simulink model "r2_b16a4x512f"  (R2012b)
settings: Solver=VariableStepDiscrete  SolverMode=SingleTasking  StartTime=0.0  StopTime=1  RelTol=1e-3
undefined symbols (not defined in the file): fft_stages, n_bits_ants, n_bits_xengs
libraries: xbsIndex_r4 x27410, casper_library_misc x230, xbsReplacements_r4 x24, casper_library_delays x8, xps_library x5, casper_library_communications x4
(part 100 of 229)

== system r2_b16a4x512f/sys0/vacc/zeros/bus_create ==
  in1 : Inport
  in2 : Inport  Port=2
  in3 : Inport  Port=3
  in4 : Inport  Port=4
  in5 : Inport  Port=5
  in6 : Inport  Port=6
  in7 : Inport  Port=7
  in8 : Inport  Port=8
  in9 : Inport  Port=9
  in10 : Inport  Port=10
  in11 : Inport  Port=11
  in12 : Inport  Port=12
  in13 : Inport  Port=13
  in14 : Inport  Port=14
  in15 : Inport  Port=15
  in16 : Inport  Port=16
  in17 : Inport  Port=17
  in18 : Inport  Port=18
  in19 : Inport  Port=19
  concatenate : xbsIndex_r4/Concat  num_inputs=19  dbl_ovrd=off  block_type=concat
  reinterpret{1..19} (19 alike) : xbsIndex_r4/Reinterpret  force_arith_type=on  arith_type=Unsigned  force_bin_pt=on  bin_pt=0  block_type=reinterpret
      reinterpret1 settings: infoedit="Changes signal type without altering the binary representation.   You can changed the signal between signed and unsigned, and relocate the binary point.<br><br>Hardware notes: In hardware this block costs nothing.<br><br>Example:  Suppose the input is 6 bits wide, signed, with 2 fractional bits, and the output is forced to unsigned with 0 fractional bits.  Then an input of -2.0 (1110.00 in binary 2's complement) becomes an output of 56 (111000 in binary)."
  bus_out : Outport
  wires:
  concatenate/1 -> bus_out/1
  in1/1 -> reinterpret1/1
  reinterpret1/1 -> concatenate/1
  in2/1 -> reinterpret2/1
  reinterpret2/1 -> concatenate/2
  in3/1 -> reinterpret3/1
  reinterpret3/1 -> concatenate/3
  in4/1 -> reinterpret4/1
  reinterpret4/1 -> concatenate/4
  in5/1 -> reinterpret5/1
  reinterpret5/1 -> concatenate/5
  in6/1 -> reinterpret6/1
  reinterpret6/1 -> concatenate/6
  in7/1 -> reinterpret7/1
  reinterpret7/1 -> concatenate/7
  in8/1 -> reinterpret8/1
  reinterpret8/1 -> concatenate/8
  in9/1 -> reinterpret9/1
  reinterpret9/1 -> concatenate/9
  in10/1 -> reinterpret10/1
  reinterpret10/1 -> concatenate/10
  in11/1 -> reinterpret11/1
  reinterpret11/1 -> concatenate/11
  in12/1 -> reinterpret12/1
  reinterpret12/1 -> concatenate/12
  in13/1 -> reinterpret13/1
  reinterpret13/1 -> concatenate/13
  in14/1 -> reinterpret14/1
  reinterpret14/1 -> concatenate/14
  in15/1 -> reinterpret15/1
  reinterpret15/1 -> concatenate/15
  in16/1 -> reinterpret16/1
  reinterpret16/1 -> concatenate/16
  in17/1 -> reinterpret17/1
  reinterpret17/1 -> concatenate/17
  in18/1 -> reinterpret18/1
  reinterpret18/1 -> concatenate/18
  in19/1 -> reinterpret19/1
  reinterpret19/1 -> concatenate/19

== system r2_b16a4x512f/sys0/vacc_tvg0/bus_replicate/bussify ==
  in1 : Inport
  in2 : Inport  Port=2
  concatenate : xbsIndex_r4/Concat  num_inputs=2  dbl_ovrd=off  block_type=concat
  reinterpret1 : xbsIndex_r4/Reinterpret  force_arith_type=on  arith_type=Unsigned  force_bin_pt=on  bin_pt=0  block_type=reinterpret
      settings: infoedit="Changes signal type without altering the binary representation.   You can changed the signal between signed and unsigned, and relocate the binary point.<br><br>Hardware notes: In hardware this block costs nothing.<br><br>Example:  Suppose the input is 6 bits wide, signed, with 2 fractional bits, and the output is forced to unsigned with 0 fractional bits.  Then an input of -2.0 (1110.00 in binary 2's complement) becomes an output of 56 (111000 in binary)."
  reinterpret2 : xbsIndex_r4/Reinterpret  force_arith_type=on  arith_type=Unsigned  force_bin_pt=on  bin_pt=0  block_type=reinterpret
      settings: infoedit="Changes signal type without altering the binary representation.   You can changed the signal between signed and unsigned, and relocate the binary point.<br><br>Hardware notes: In hardware this block costs nothing.<br><br>Example:  Suppose the input is 6 bits wide, signed, with 2 fractional bits, and the output is forced to unsigned with 0 fractional bits.  Then an input of -2.0 (1110.00 in binary 2's complement) becomes an output of 56 (111000 in binary)."
  bus_out : Outport
  wires:
  concatenate/1 -> bus_out/1
  in1/1 -> reinterpret1/1
  reinterpret1/1 -> concatenate/1
  in2/1 -> reinterpret2/1
  reinterpret2/1 -> concatenate/2

== system r2_b16a4x512f/sys0/vacc_tvg0/bus_replicate1/bussify ==
  in1 : Inport
  in2 : Inport  Port=2
  concatenate : xbsIndex_r4/Concat  num_inputs=2  dbl_ovrd=off  block_type=concat
  reinterpret1 : xbsIndex_r4/Reinterpret  force_arith_type=on  arith_type=Unsigned  force_bin_pt=on  bin_pt=0  block_type=reinterpret
      settings: infoedit="Changes signal type without altering the binary representation.   You can changed the signal between signed and unsigned, and relocate the binary point.<br><br>Hardware notes: In hardware this block costs nothing.<br><br>Example:  Suppose the input is 6 bits wide, signed, with 2 fractional bits, and the output is forced to unsigned with 0 fractional bits.  Then an input of -2.0 (1110.00 in binary 2's complement) becomes an output of 56 (111000 in binary)."
  reinterpret2 : xbsIndex_r4/Reinterpret  force_arith_type=on  arith_type=Unsigned  force_bin_pt=on  bin_pt=0  block_type=reinterpret
      settings: infoedit="Changes signal type without altering the binary representation.   You can changed the signal between signed and unsigned, and relocate the binary point.<br><br>Hardware notes: In hardware this block costs nothing.<br><br>Example:  Suppose the input is 6 bits wide, signed, with 2 fractional bits, and the output is forced to unsigned with 0 fractional bits.  Then an input of -2.0 (1110.00 in binary 2's complement) becomes an output of 56 (111000 in binary)."
  bus_out : Outport
  wires:
  reinterpret2/1 -> concatenate/2
  in2/1 -> reinterpret2/1
  reinterpret1/1 -> concatenate/1
  in1/1 -> reinterpret1/1
  concatenate/1 -> bus_out/1

== system r2_b16a4x512f/sys0/vacc_tvg0/generate_pulses/edge_detect ==
  in : Inport
  Delay : xbsIndex_r4/Delay  rst=off  infoeditControl=Selection of Reset will increase slice count due to use of real FFs and instead of SRLs  en=off  latency=1  dbl_ovrd=off  reg_retiming=on  block_type=delay
      settings: xl_area=[0, 0, 0, 0, 0, 0, 0]
  Inverter : xbsIndex_r4/Inverter  en=off  latency=0  dbl_ovrd=off  block_type=inv
      settings: xl_area=[0, 0, 0, 0, 0, 0, 0]
  edge_op : xbsIndex_r4/Logical  logical_function=NOR  inputs=2  en=off  latency=0  precision=Full  arith_type=Unsigned  n_bits=8  bin_pt=2  align_bp=on  dbl_ovrd=off  block_type=logical
      settings: xl_area=[0, 0, 0, 0, 0, 0, 0]
  out : Outport
  wires:
  Delay/1 -> edge_op/2
  in/1 -> Delay/1, Inverter/1
  edge_op/1 -> out/1
  Inverter/1 -> edge_op/1

== system r2_b16a4x512f/sys0/vacc_tvg0/generate_pulses/edge_detect1 ==
  in : Inport
  Delay : xbsIndex_r4/Delay  rst=off  infoeditControl=Selection of Reset will increase slice count due to use of real FFs and instead of SRLs  en=off  latency=1  dbl_ovrd=off  reg_retiming=on  block_type=delay
      settings: xl_area=[0, 0, 0, 0, 0, 0, 0]
  Inverter : xbsIndex_r4/Inverter  en=off  latency=0  dbl_ovrd=off  block_type=inv
      settings: xl_area=[0, 0, 0, 0, 0, 0, 0]
  edge_op : xbsIndex_r4/Logical  logical_function=XNOR  inputs=2  en=off  latency=0  precision=Full  arith_type=Unsigned  n_bits=8  bin_pt=2  align_bp=on  dbl_ovrd=off  block_type=logical
      settings: xl_area=[0, 0, 0, 0, 0, 0, 0]
  out : Outport
  wires:
  Inverter/1 -> edge_op/1
  edge_op/1 -> out/1
  in/1 -> Inverter/1, Delay/1
  Delay/1 -> edge_op/2

== system r2_b16a4x512f/sys0/vacc_tvg0/ins_counter/bus_replicate1 ==
  in : Inport
  bussify : Subsystem  AncestorBlock=casper_library_flow_control/bus_create  mask(bus_create){inputNum=2}
      mask prompts: inputNum "Number of inputs:"
      mask init:
      | bus_create_init(gcb,...
      |     'inputNum', inputNum);
  out : Outport
  wires:
  in/1 -> bussify/1(in1), bussify/2(in2)
  bussify/1(bus_out) -> out/1

== system r2_b16a4x512f/sys0/xeng/auto_tap/delay ==
  din : Inport
  constant : xbsIndex_r4/Constant  const=1  gui_display_data_type=Fixed-point  arith_type=Boolean  n_bits=16  bin_pt=14  preci_type=Single  exp_width=8  frac_width=24  explicit_period=on  period=1  equ=P=C  opselect=C  inp2=PCIN>>17  opr=+  inp1=P  carry=CIN  dbl_ovrd=off  block_type=constant
  counter : xbsIndex_r4/Counter  cnt_type=Count Limited  cnt_to=DelayLen - bram_latency - 1  operation=Up  start_count=0  cnt_by_val=1  arith_type=Unsigned  n_bits=11  bin_pt=0  load_pin=off  rst=off  en=off  explicit_period=on  period=1  dbl_ovrd=off  use_behavioral_HDL=off  implementation=Fabric  use_rpm=off  block_type=counter
  ram : xbsIndex_r4/Single Port RAM  depth=2048  initVector=0  distributed_mem=Block RAM  write_mode=Read Before Write  rst=off  init_reg=0  en=off  latency=bram_latency  dbl_ovrd=off  optimize=Area  block_type=spram
  dout : Outport
  wires:
  counter/1 -> ram/1
  din/1 -> ram/2
  constant/1 -> ram/3
  ram/1 -> dout/1

== system r2_b16a4x512f/sys0/xeng/auto_tap/dual_pol_cmac ==
  a1 : Inport
  a2 : Inport  Port=2
  acc_in : Inport  Port=3
  sync : Inport  Port=4
  valid_in : Inport  Port=5
  Concat : xbsIndex_r4/Concat  num_inputs=4  dbl_ovrd=off  block_type=concat
      settings: block_version=9.2.01
  Constant1 : xbsIndex_r4/Constant  const=0  gui_display_data_type=Fixed-point  arith_type=Unsigned  n_bits=1  bin_pt=0  preci_type=Single  exp_width=8  frac_width=24  explicit_period=on  period=1  equ=P=C  opselect=C  inp2=PCIN>>17  opr=+  inp1=P  carry=CIN  dbl_ovrd=off  block_type=constant
      settings: block_version=9.2.01
  Constant2 : xbsIndex_r4/Constant  const=0  gui_display_data_type=Fixed-point  arith_type=Unsigned  n_bits=1  bin_pt=0  preci_type=Single  exp_width=8  frac_width=24  explicit_period=on  period=1  equ=P=C  opselect=C  inp2=PCIN>>17  opr=+  inp1=P  carry=CIN  dbl_ovrd=off  block_type=constant
      settings: block_version=9.2.01
  Constant4 : xbsIndex_r4/Constant  const=0  gui_display_data_type=Fixed-point  arith_type=Unsigned  n_bits=1  bin_pt=0  preci_type=Single  exp_width=8  frac_width=24  explicit_period=on  period=1  equ=P=C  opselect=C  inp2=PCIN>>17  opr=+  inp1=P  carry=CIN  dbl_ovrd=off  block_type=constant
      settings: block_version=9.2.01
  Slice{,1,6,10} (4 alike) : xbsIndex_r4/Slice  nbits=2*n_bits  boolean_output=off  mode=Upper Bit Location + Width  bit1=0  base1=MSB of Input  bit0=0  base0=LSB of Input  dbl_ovrd=off  block_type=slice
      Slice settings: infoedit="Extracts a given range of bits from each input sample and presents it at the output.  The output type is ordinarily unsigned with binary point at zero, but can be Boolean when the slice is one bit wide.<P><P>Hardware notes: In hardware this block costs nothing."  block_version=9.2.01
      Slice1 settings: infoedit="Extracts a given range of bits from each input sample and presents it at the output.  The output type is ordinarily unsigned with binary point at zero, but can be Boolean when the slice is one bit wide.<P><P>Hardware notes: In hardware this block costs nothing."  block_version=9.2.01
      Slice10 settings: block_version=9.2.01
      Slice6 settings: infoedit="Extracts a given range of bits from each input sample and presents it at the output.  The output type is ordinarily unsigned with binary point at zero, but can be Boolean when the slice is one bit wide.<P><P>Hardware notes: In hardware this block costs nothing."  block_version=9.2.01
  Slice11 : xbsIndex_r4/Slice  nbits=2*n_bits_out  boolean_output=off  mode=Upper Bit Location + Width  bit1=-6*n_bits_out  base1=MSB of Input  bit0=0  base0=LSB of Input  dbl_ovrd=off  block_type=slice
      settings: infoedit="Extracts a given range of bits from each input sample and presents it at the output.  The output type is ordinarily unsigned with binary point at zero, but can be Boolean when the slice is one bit wide.<P><P>Hardware notes: In hardware this block costs nothing."  block_version=9.2.01
  Slice2 : xbsIndex_r4/Slice  nbits=2*n_bits_out  boolean_output=off  mode=Upper Bit Location + Width  bit1=0  base1=MSB of Input  bit0=0  base0=LSB of Input  dbl_ovrd=off  block_type=slice
      settings: infoedit="Extracts a given range of bits from each input sample and presents it at the output.  The output type is ordinarily unsigned with binary point at zero, but can be Boolean when the slice is one bit wide.<P><P>Hardware notes: In hardware this block costs nothing."  block_version=9.2.01
  Slice{3..4,7,9} (4 alike) : xbsIndex_r4/Slice  nbits=2*n_bits  boolean_output=off  mode=Upper Bit Location + Width  bit1=-2*n_bits  base1=MSB of Input  bit0=0  base0=LSB of Input  dbl_ovrd=off  block_type=slice
      Slice3 settings: infoedit="Extracts a given range of bits from each input sample and presents it at the output.  The output type is ordinarily unsigned with binary point at zero, but can be Boolean when the slice is one bit wide.<P><P>Hardware notes: In hardware this block costs nothing."  block_version=9.2.01
      Slice4 settings: infoedit="Extracts a given range of bits from each input sample and presents it at the output.  The output type is ordinarily unsigned with binary point at zero, but can be Boolean when the slice is one bit wide.<P><P>Hardware notes: In hardware this block costs nothing."  block_version=9.2.01
      Slice7 settings: infoedit="Extracts a given range of bits from each input sample and presents it at the output.  The output type is ordinarily unsigned with binary point at zero, but can be Boolean when the slice is one bit wide.<P><P>Hardware notes: In hardware this block costs nothing."  block_version=9.2.01
      Slice9 settings: block_version=9.2.01
  Slice5 : xbsIndex_r4/Slice  nbits=2*n_bits_out  boolean_output=off  mode=Upper Bit Location + Width  bit1=-2*n_bits_out  base1=MSB of Input  bit0=0  base0=LSB of Input  dbl_ovrd=off  block_type=slice
      settings: infoedit="Extracts a given range of bits from each input sample and presents it at the output.  The output type is ordinarily unsigned with binary point at zero, but can be Boolean when the slice is one bit wide.<P><P>Hardware notes: In hardware this block costs nothing."  block_version=9.2.01
  Slice8 : xbsIndex_r4/Slice  nbits=2*n_bits_out  boolean_output=off  mode=Upper Bit Location + Width  bit1=-4*n_bits_out  base1=MSB of Input  bit0=0  base0=LSB of Input  dbl_ovrd=off  block_type=slice
      settings: infoedit="Extracts a given range of bits from each input sample and presents it at the output.  The output type is ordinarily unsigned with binary point at zero, but can be Boolean when the slice is one bit wide.<P><P>Hardware notes: In hardware this block costs nothing."  block_version=9.2.01
  Terminator : Terminator
  Terminator1 : Terminator
  Terminator2 : Terminator
  cmac1 : Subsystem  Tag=cmac  AncestorBlock=casper_library_correlator/cmac  mask(cmac){acc_len=256, n_bits_a=8, bin_pt_a=7, n_bits_b=8, bin_pt_b=7, quantization=Truncate, overflow=Wrap, mult_latency=4, add_latency=3, in_latency=0, conv_latency=0, multiplier_implementation=embedded multiplier core}
      mask prompts: acc_len "Number of Accumulations"; n_bits_a "Number of bits 'a'"; bin_pt_a "Binary point 'a'"; n_bits_b "Number of bits 'b'"; bin_pt_b "Binary point 'b'"; quantization "Quantisation"; mult_latency "Multiplier Latency"; add_latency "Adder Latency"; in_latency "Input Latency"; conv_latency "Convert Latency"; multiplier_implementation "Multiplier Implementation"
      mask help: A complex multiply-accumulate block. Full precision.
      mask init:
      | bit_growth = ceil(log2(acc_len));
      | n_bits_out = (n_bits_a + n_bits_b + 1 + bit_growth);
      | bin_pt_out=(bin_pt_a + bin_pt_b);
      | set_param([gcb,'/cmult*'],'multiplier_implementation',num2str(multiplier_implementation));
      | set_param([gcb,'/cmult*'],'mult_latency',num2str(mult_latency));
      | set_param([gcb,'/cmult*'],'conjugated','on');
      | set_param([gcb,'/cmult*'],'add_latency',num2str(add_latency));
      | set_param([gcb,'/cmult*'],'n_bits_ab',num2str(n_bits_out));
      | set_param([gcb,'/cmult*'],'n_bits_a',num2str(n_bits_a));
      | set_param([gcb,'/cmult*'],'n_bits_b',num2str(n_bits_b));
      | set_param([gcb,'/cmult*'],'bin_pt_a',num2str(bin_pt_a));
      | set_param([gcb,'/cmult*'],'bin_pt_b',num2str(bin_pt_b));
      | set_param([gcb,'/cmult*'],'bin_pt_ab',num2str(bin_pt_out));
      mask TypeOptions quantization: Truncate | Round  (unbiased: +/- Inf) | Round  (unbiased: Even Values)
      mask TypeOptions overflow: Wrap | Saturate | Flag as error
      mask TypeOptions multiplier_implementation: behavioral HDL | standard core | embedded multiplier core
  cmac2 : Subsystem  Tag=cmac  AncestorBlock=casper_library_correlator/cmac  mask(cmac){acc_len=256, n_bits_a=8, bin_pt_a=7, n_bits_b=8, bin_pt_b=7, quantization=Truncate, overflow=Wrap, mult_latency=4, add_latency=3, in_latency=0, conv_latency=0, multiplier_implementation=embedded multiplier core}
      mask prompts: acc_len "Number of Accumulations"; n_bits_a "Number of bits 'a'"; bin_pt_a "Binary point 'a'"; n_bits_b "Number of bits 'b'"; bin_pt_b "Binary point 'b'"; quantization "Quantisation"; mult_latency "Multiplier Latency"; add_latency "Adder Latency"; in_latency "Input Latency"; conv_latency "Convert Latency"; multiplier_implementation "Multiplier Implementation"
      mask help: A complex multiply-accumulate block. Full precision.
      mask init: same as r2_b16a4x512f/sys0/xeng/auto_tap/dual_pol_cmac/cmac1
      mask TypeOptions quantization: Truncate | Round  (unbiased: +/- Inf) | Round  (unbiased: Even Values)
      mask TypeOptions overflow: Wrap | Saturate | Flag as error
      mask TypeOptions multiplier_implementation: behavioral HDL | standard core | embedded multiplier core
  cmac3 : Subsystem  Tag=cmac  AncestorBlock=casper_library_correlator/cmac  mask(cmac){acc_len=256, n_bits_a=8, bin_pt_a=7, n_bits_b=8, bin_pt_b=7, quantization=Truncate, overflow=Wrap, mult_latency=4, add_latency=3, in_latency=0, conv_latency=0, multiplier_implementation=embedded multiplier core}
      mask prompts: acc_len "Number of Accumulations"; n_bits_a "Number of bits 'a'"; bin_pt_a "Binary point 'a'"; n_bits_b "Number of bits 'b'"; bin_pt_b "Binary point 'b'"; quantization "Quantisation"; mult_latency "Multiplier Latency"; add_latency "Adder Latency"; in_latency "Input Latency"; conv_latency "Convert Latency"; multiplier_implementation "Multiplier Implementation"
      mask help: A complex multiply-accumulate block. Full precision.
      mask init: same as r2_b16a4x512f/sys0/xeng/auto_tap/dual_pol_cmac/cmac1
      mask TypeOptions quantization: Truncate | Round  (unbiased: +/- Inf) | Round  (unbiased: Even Values)
      mask TypeOptions overflow: Wrap | Saturate | Flag as error
      mask TypeOptions multiplier_implementation: behavioral HDL | standard core | embedded multiplier core
  cmac4 : Subsystem  Tag=cmac  AncestorBlock=casper_library_correlator/cmac  mask(cmac){acc_len=256, n_bits_a=8, bin_pt_a=7, n_bits_b=8, bin_pt_b=7, quantization=Truncate, overflow=Wrap, mult_latency=4, add_latency=3, in_latency=0, conv_latency=0, multiplier_implementation=embedded multiplier core}
      mask prompts: acc_len "Number of Accumulations"; n_bits_a "Number of bits 'a'"; bin_pt_a "Binary point 'a'"; n_bits_b "Number of bits 'b'"; bin_pt_b "Binary point 'b'"; quantization "Quantisation"; mult_latency "Multiplier Latency"; add_latency "Adder Latency"; in_latency "Input Latency"; conv_latency "Convert Latency"; multiplier_implementation "Multiplier Implementation"
      mask help: A complex multiply-accumulate block. Full precision.
      mask init: same as r2_b16a4x512f/sys0/xeng/auto_tap/dual_pol_cmac/cmac1
      mask TypeOptions quantization: Truncate | Round  (unbiased: +/- Inf) | Round  (unbiased: Even Values)
      mask TypeOptions overflow: Wrap | Saturate | Flag as error
      mask TypeOptions multiplier_implementation: behavioral HDL | standard core | embedded multiplier core
  acc_out : Outport
  valid_out : Outport  Port=2
  wires:
  acc_in/1 -> Slice2/1, Slice5/1, Slice8/1, Slice11/1
  a2/1 -> Slice10/1, Slice7/1, Slice4/1, Slice1/1
  a1/1 -> Slice9/1, Slice6/1, Slice3/1, Slice/1
  cmac4/1(acc_out) -> Concat/4
  cmac3/1(acc_out) -> Concat/3
  cmac2/1(acc_out) -> Concat/2
  cmac1/1(acc_out) -> Concat/1
  cmac4/2(valid_out) -> valid_out/1
  cmac3/2(valid_out) -> Terminator2/1
  cmac2/2(valid_out) -> Terminator1/1
  sync/1 -> cmac4/4(sync), cmac3/4(sync), cmac2/4(sync), cmac1/4(sync)
  Slice11/1 -> cmac4/3(acc_in)
  Slice10/1 -> cmac4/2(c+di)
  Slice9/1 -> cmac4/1(a+bi)
  Constant4/1 -> cmac3/5(valid_in)
  Slice8/1 -> cmac3/3(acc_in)
  Slice7/1 -> cmac3/2(c+di)
  Slice6/1 -> cmac3/1(a+bi)
  Constant1/1 -> cmac2/5(valid_in)
  cmac1/2(valid_out) -> Terminator/1
  valid_in/1 -> cmac4/5(valid_in)
  Concat/1 -> acc_out/1
  Slice5/1 -> cmac2/3(acc_in)
  Slice4/1 -> cmac2/2(c+di)
  Slice3/1 -> cmac2/1(a+bi)
  Slice2/1 -> cmac1/3(acc_in)
  Slice1/1 -> cmac1/2(c+di)
  Slice/1 -> cmac1/1(a+bi)
  Constant2/1 -> cmac1/5(valid_in)

== system r2_b16a4x512f/sys0/xeng/baseline_tap1/delay ==
  din : Inport
  constant : xbsIndex_r4/Constant  const=1  gui_display_data_type=Fixed-point  arith_type=Boolean  n_bits=16  bin_pt=14  preci_type=Single  exp_width=8  frac_width=24  explicit_period=on  period=1  equ=P=C  opselect=C  inp2=PCIN>>17  opr=+  inp1=P  carry=CIN  dbl_ovrd=off  block_type=constant
  counter : xbsIndex_r4/Counter  cnt_type=Count Limited  cnt_to=DelayLen - bram_latency - 1  operation=Up  start_count=0  cnt_by_val=1  arith_type=Unsigned  n_bits=8  bin_pt=0  load_pin=off  rst=off  en=off  explicit_period=on  period=1  dbl_ovrd=off  use_behavioral_HDL=off  implementation=Fabric  use_rpm=off  block_type=counter
  ram : xbsIndex_r4/Single Port RAM  depth=256  initVector=0  distributed_mem=Block RAM  write_mode=Read Before Write  rst=off  init_reg=0  en=off  latency=bram_latency  dbl_ovrd=off  optimize=Area  block_type=spram
  dout : Outport
  wires:
  counter/1 -> ram/1
  din/1 -> ram/2
  constant/1 -> ram/3
  ram/1 -> dout/1

== system r2_b16a4x512f/sys0/xeng/baseline_tap1/dual_pol_cmac ==
  a1 : Inport
  a2 : Inport  Port=2
  acc_in : Inport  Port=3
  sync : Inport  Port=4
  valid_in : Inport  Port=5
  Concat : xbsIndex_r4/Concat  num_inputs=4  dbl_ovrd=off  block_type=concat
      settings: block_version=9.2.01
  Constant1 : xbsIndex_r4/Constant  const=0  gui_display_data_type=Fixed-point  arith_type=Unsigned  n_bits=1  bin_pt=0  preci_type=Single  exp_width=8  frac_width=24  explicit_period=on  period=1  equ=P=C  opselect=C  inp2=PCIN>>17  opr=+  inp1=P  carry=CIN  dbl_ovrd=off  block_type=constant
      settings: block_version=9.2.01
  Constant2 : xbsIndex_r4/Constant  const=0  gui_display_data_type=Fixed-point  arith_type=Unsigned  n_bits=1  bin_pt=0  preci_type=Single  exp_width=8  frac_width=24  explicit_period=on  period=1  equ=P=C  opselect=C  inp2=PCIN>>17  opr=+  inp1=P  carry=CIN  dbl_ovrd=off  block_type=constant
      settings: block_version=9.2.01
  Constant4 : xbsIndex_r4/Constant  const=0  gui_display_data_type=Fixed-point  arith_type=Unsigned  n_bits=1  bin_pt=0  preci_type=Single  exp_width=8  frac_width=24  explicit_period=on  period=1  equ=P=C  opselect=C  inp2=PCIN>>17  opr=+  inp1=P  carry=CIN  dbl_ovrd=off  block_type=constant
      settings: block_version=9.2.01
  Slice{,1,6,10} (4 alike) : xbsIndex_r4/Slice  nbits=2*n_bits  boolean_output=off  mode=Upper Bit Location + Width  bit1=0  base1=MSB of Input  bit0=0  base0=LSB of Input  dbl_ovrd=off  block_type=slice
      Slice settings: infoedit="Extracts a given range of bits from each input sample and presents it at the output.  The output type is ordinarily unsigned with binary point at zero, but can be Boolean when the slice is one bit wide.<P><P>Hardware notes: In hardware this block costs nothing."  block_version=9.2.01
      Slice1 settings: infoedit="Extracts a given range of bits from each input sample and presents it at the output.  The output type is ordinarily unsigned with binary point at zero, but can be Boolean when the slice is one bit wide.<P><P>Hardware notes: In hardware this block costs nothing."  block_version=9.2.01
      Slice10 settings: block_version=9.2.01
      Slice6 settings: infoedit="Extracts a given range of bits from each input sample and presents it at the output.  The output type is ordinarily unsigned with binary point at zero, but can be Boolean when the slice is one bit wide.<P><P>Hardware notes: In hardware this block costs nothing."  block_version=9.2.01
  Slice11 : xbsIndex_r4/Slice  nbits=2*n_bits_out  boolean_output=off  mode=Upper Bit Location + Width  bit1=-6*n_bits_out  base1=MSB of Input  bit0=0  base0=LSB of Input  dbl_ovrd=off  block_type=slice
      settings: infoedit="Extracts a given range of bits from each input sample and presents it at the output.  The output type is ordinarily unsigned with binary point at zero, but can be Boolean when the slice is one bit wide.<P><P>Hardware notes: In hardware this block costs nothing."  block_version=9.2.01
  Slice2 : xbsIndex_r4/Slice  nbits=2*n_bits_out  boolean_output=off  mode=Upper Bit Location + Width  bit1=0  base1=MSB of Input  bit0=0  base0=LSB of Input  dbl_ovrd=off  block_type=slice
      settings: infoedit="Extracts a given range of bits from each input sample and presents it at the output.  The output type is ordinarily unsigned with binary point at zero, but can be Boolean when the slice is one bit wide.<P><P>Hardware notes: In hardware this block costs nothing."  block_version=9.2.01
  Slice{3..4,7,9} (4 alike) : xbsIndex_r4/Slice  nbits=2*n_bits  boolean_output=off  mode=Upper Bit Location + Width  bit1=-2*n_bits  base1=MSB of Input  bit0=0  base0=LSB of Input  dbl_ovrd=off  block_type=slice
      Slice3 settings: infoedit="Extracts a given range of bits from each input sample and presents it at the output.  The output type is ordinarily unsigned with binary point at zero, but can be Boolean when the slice is one bit wide.<P><P>Hardware notes: In hardware this block costs nothing."  block_version=9.2.01
      Slice4 settings: infoedit="Extracts a given range of bits from each input sample and presents it at the output.  The output type is ordinarily unsigned with binary point at zero, but can be Boolean when the slice is one bit wide.<P><P>Hardware notes: In hardware this block costs nothing."  block_version=9.2.01
      Slice7 settings: infoedit="Extracts a given range of bits from each input sample and presents it at the output.  The output type is ordinarily unsigned with binary point at zero, but can be Boolean when the slice is one bit wide.<P><P>Hardware notes: In hardware this block costs nothing."  block_version=9.2.01
      Slice9 settings: block_version=9.2.01
  Slice5 : xbsIndex_r4/Slice  nbits=2*n_bits_out  boolean_output=off  mode=Upper Bit Location + Width  bit1=-2*n_bits_out  base1=MSB of Input  bit0=0  base0=LSB of Input  dbl_ovrd=off  block_type=slice
      settings: infoedit="Extracts a given range of bits from each input sample and presents it at the output.  The output type is ordinarily unsigned with binary point at zero, but can be Boolean when the slice is one bit wide.<P><P>Hardware notes: In hardware this block costs nothing."  block_version=9.2.01
  Slice8 : xbsIndex_r4/Slice  nbits=2*n_bits_out  boolean_output=off  mode=Upper Bit Location + Width  bit1=-4*n_bits_out  base1=MSB of Input  bit0=0  base0=LSB of Input  dbl_ovrd=off  block_type=slice
      settings: infoedit="Extracts a given range of bits from each input sample and presents it at the output.  The output type is ordinarily unsigned with binary point at zero, but can be Boolean when the slice is one bit wide.<P><P>Hardware notes: In hardware this block costs nothing."  block_version=9.2.01
  Terminator : Terminator
  Terminator1 : Terminator
  Terminator2 : Terminator
  cmac1 : Subsystem  Tag=cmac  AncestorBlock=casper_library_correlator/cmac  mask(cmac){acc_len=256, n_bits_a=8, bin_pt_a=7, n_bits_b=8, bin_pt_b=7, quantization=Truncate, overflow=Wrap, mult_latency=4, add_latency=3, in_latency=0, conv_latency=0, multiplier_implementation=embedded multiplier core}
      mask prompts: acc_len "Number of Accumulations"; n_bits_a "Number of bits 'a'"; bin_pt_a "Binary point 'a'"; n_bits_b "Number of bits 'b'"; bin_pt_b "Binary point 'b'"; quantization "Quantisation"; mult_latency "Multiplier Latency"; add_latency "Adder Latency"; in_latency "Input Latency"; conv_latency "Convert Latency"; multiplier_implementation "Multiplier Implementation"
      mask help: A complex multiply-accumulate block. Full precision.
      mask init: same as r2_b16a4x512f/sys0/xeng/auto_tap/dual_pol_cmac/cmac1
      mask TypeOptions quantization: Truncate | Round  (unbiased: +/- Inf) | Round  (unbiased: Even Values)
      mask TypeOptions overflow: Wrap | Saturate | Flag as error
      mask TypeOptions multiplier_implementation: behavioral HDL | standard core | embedded multiplier core
  cmac2 : Subsystem  Tag=cmac  AncestorBlock=casper_library_correlator/cmac  mask(cmac){acc_len=256, n_bits_a=8, bin_pt_a=7, n_bits_b=8, bin_pt_b=7, quantization=Truncate, overflow=Wrap, mult_latency=4, add_latency=3, in_latency=0, conv_latency=0, multiplier_implementation=embedded multiplier core}
      mask prompts: acc_len "Number of Accumulations"; n_bits_a "Number of bits 'a'"; bin_pt_a "Binary point 'a'"; n_bits_b "Number of bits 'b'"; bin_pt_b "Binary point 'b'"; quantization "Quantisation"; mult_latency "Multiplier Latency"; add_latency "Adder Latency"; in_latency "Input Latency"; conv_latency "Convert Latency"; multiplier_implementation "Multiplier Implementation"
      mask help: A complex multiply-accumulate block. Full precision.
      mask init: same as r2_b16a4x512f/sys0/xeng/auto_tap/dual_pol_cmac/cmac1
      mask TypeOptions quantization: Truncate | Round  (unbiased: +/- Inf) | Round  (unbiased: Even Values)
      mask TypeOptions overflow: Wrap | Saturate | Flag as error
      mask TypeOptions multiplier_implementation: behavioral HDL | standard core | embedded multiplier core
  cmac3 : Subsystem  Tag=cmac  AncestorBlock=casper_library_correlator/cmac  mask(cmac){acc_len=256, n_bits_a=8, bin_pt_a=7, n_bits_b=8, bin_pt_b=7, quantization=Truncate, overflow=Wrap, mult_latency=4, add_latency=3, in_latency=0, conv_latency=0, multiplier_implementation=embedded multiplier core}
      mask prompts: acc_len "Number of Accumulations"; n_bits_a "Number of bits 'a'"; bin_pt_a "Binary point 'a'"; n_bits_b "Number of bits 'b'"; bin_pt_b "Binary point 'b'"; quantization "Quantisation"; mult_latency "Multiplier Latency"; add_latency "Adder Latency"; in_latency "Input Latency"; conv_latency "Convert Latency"; multiplier_implementation "Multiplier Implementation"
      mask help: A complex multiply-accumulate block. Full precision.
      mask init: same as r2_b16a4x512f/sys0/xeng/auto_tap/dual_pol_cmac/cmac1
      mask TypeOptions quantization: Truncate | Round  (unbiased: +/- Inf) | Round  (unbiased: Even Values)
      mask TypeOptions overflow: Wrap | Saturate | Flag as error
      mask TypeOptions multiplier_implementation: behavioral HDL | standard core | embedded multiplier core
  cmac4 : Subsystem  Tag=cmac  AncestorBlock=casper_library_correlator/cmac  mask(cmac){acc_len=256, n_bits_a=8, bin_pt_a=7, n_bits_b=8, bin_pt_b=7, quantization=Truncate, overflow=Wrap, mult_latency=4, add_latency=3, in_latency=0, conv_latency=0, multiplier_implementation=embedded multiplier core}
      mask prompts: acc_len "Number of Accumulations"; n_bits_a "Number of bits 'a'"; bin_pt_a "Binary point 'a'"; n_bits_b "Number of bits 'b'"; bin_pt_b "Binary point 'b'"; quantization "Quantisation"; mult_latency "Multiplier Latency"; add_latency "Adder Latency"; in_latency "Input Latency"; conv_latency "Convert Latency"; multiplier_implementation "Multiplier Implementation"
      mask help: A complex multiply-accumulate block. Full precision.
      mask init: same as r2_b16a4x512f/sys0/xeng/auto_tap/dual_pol_cmac/cmac1
      mask TypeOptions quantization: Truncate | Round  (unbiased: +/- Inf) | Round  (unbiased: Even Values)
      mask TypeOptions overflow: Wrap | Saturate | Flag as error
      mask TypeOptions multiplier_implementation: behavioral HDL | standard core | embedded multiplier core
  acc_out : Outport
  valid_out : Outport  Port=2
  wires:
  acc_in/1 -> Slice2/1, Slice5/1, Slice8/1, Slice11/1
  a2/1 -> Slice10/1, Slice7/1, Slice4/1, Slice1/1
  a1/1 -> Slice9/1, Slice6/1, Slice3/1, Slice/1
  cmac4/1(acc_out) -> Concat/4
  cmac3/1(acc_out) -> Concat/3
  cmac2/1(acc_out) -> Concat/2
  cmac1/1(acc_out) -> Concat/1
  cmac4/2(valid_out) -> valid_out/1
  cmac3/2(valid_out) -> Terminator2/1
  cmac2/2(valid_out) -> Terminator1/1
  sync/1 -> cmac4/4(sync), cmac3/4(sync), cmac2/4(sync), cmac1/4(sync)
  Slice11/1 -> cmac4/3(acc_in)
  Slice10/1 -> cmac4/2(c+di)
  Slice9/1 -> cmac4/1(a+bi)
  Constant4/1 -> cmac3/5(valid_in)
  Slice8/1 -> cmac3/3(acc_in)
  Slice7/1 -> cmac3/2(c+di)
  Slice6/1 -> cmac3/1(a+bi)
  Constant1/1 -> cmac2/5(valid_in)
  cmac1/2(valid_out) -> Terminator/1
  valid_in/1 -> cmac4/5(valid_in)
  Concat/1 -> acc_out/1
  Slice5/1 -> cmac2/3(acc_in)
  Slice4/1 -> cmac2/2(c+di)
  Slice3/1 -> cmac2/1(a+bi)
  Slice2/1 -> cmac1/3(acc_in)
  Slice1/1 -> cmac1/2(c+di)
  Slice/1 -> cmac1/1(a+bi)
  Constant2/1 -> cmac1/5(valid_in)

== system r2_b16a4x512f/sys0/xeng/baseline_tap2/delay ==
  din : Inport
  constant : xbsIndex_r4/Constant  const=1  gui_display_data_type=Fixed-point  arith_type=Boolean  n_bits=16  bin_pt=14  preci_type=Single  exp_width=8  frac_width=24  explicit_period=on  period=1  equ=P=C  opselect=C  inp2=PCIN>>17  opr=+  inp1=P  carry=CIN  dbl_ovrd=off  block_type=constant
  counter : xbsIndex_r4/Counter  cnt_type=Count Limited  cnt_to=DelayLen - bram_latency - 1  operation=Up  start_count=0  cnt_by_val=1  arith_type=Unsigned  n_bits=8  bin_pt=0  load_pin=off  rst=off  en=off  explicit_period=on  period=1  dbl_ovrd=off  use_behavioral_HDL=off  implementation=Fabric  use_rpm=off  block_type=counter
  ram : xbsIndex_r4/Single Port RAM  depth=256  initVector=0  distributed_mem=Block RAM  write_mode=Read Before Write  rst=off  init_reg=0  en=off  latency=bram_latency  dbl_ovrd=off  optimize=Area  block_type=spram
  dout : Outport
  wires:
  counter/1 -> ram/1
  din/1 -> ram/2
  constant/1 -> ram/3
  ram/1 -> dout/1

== system r2_b16a4x512f/sys0/xeng/baseline_tap2/dual_pol_cmac ==
  a1 : Inport
  a2 : Inport  Port=2
  acc_in : Inport  Port=3
  sync : Inport  Port=4
  valid_in : Inport  Port=5
  Concat : xbsIndex_r4/Concat  num_inputs=4  dbl_ovrd=off  block_type=concat
      settings: block_version=9.2.01
  Constant1 : xbsIndex_r4/Constant  const=0  gui_display_data_type=Fixed-point  arith_type=Unsigned  n_bits=1  bin_pt=0  preci_type=Single  exp_width=8  frac_width=24  explicit_period=on  period=1  equ=P=C  opselect=C  inp2=PCIN>>17  opr=+  inp1=P  carry=CIN  dbl_ovrd=off  block_type=constant
      settings: block_version=9.2.01
  Constant2 : xbsIndex_r4/Constant  const=0  gui_display_data_type=Fixed-point  arith_type=Unsigned  n_bits=1  bin_pt=0  preci_type=Single  exp_width=8  frac_width=24  explicit_period=on  period=1  equ=P=C  opselect=C  inp2=PCIN>>17  opr=+  inp1=P  carry=CIN  dbl_ovrd=off  block_type=constant
      settings: block_version=9.2.01
  Constant4 : xbsIndex_r4/Constant  const=0  gui_display_data_type=Fixed-point  arith_type=Unsigned  n_bits=1  bin_pt=0  preci_type=Single  exp_width=8  frac_width=24  explicit_period=on  period=1  equ=P=C  opselect=C  inp2=PCIN>>17  opr=+  inp1=P  carry=CIN  dbl_ovrd=off  block_type=constant
      settings: block_version=9.2.01
  Slice{,1,6,10} (4 alike) : xbsIndex_r4/Slice  nbits=2*n_bits  boolean_output=off  mode=Upper Bit Location + Width  bit1=0  base1=MSB of Input  bit0=0  base0=LSB of Input  dbl_ovrd=off  block_type=slice
      Slice settings: infoedit="Extracts a given range of bits from each input sample and presents it at the output.  The output type is ordinarily unsigned with binary point at zero, but can be Boolean when the slice is one bit wide.<P><P>Hardware notes: In hardware this block costs nothing."  block_version=9.2.01
      Slice1 settings: infoedit="Extracts a given range of bits from each input sample and presents it at the output.  The output type is ordinarily unsigned with binary point at zero, but can be Boolean when the slice is one bit wide.<P><P>Hardware notes: In hardware this block costs nothing."  block_version=9.2.01
      Slice10 settings: block_version=9.2.01
      Slice6 settings: infoedit="Extracts a given range of bits from each input sample and presents it at the output.  The output type is ordinarily unsigned with binary point at zero, but can be Boolean when the slice is one bit wide.<P><P>Hardware notes: In hardware this block costs nothing."  block_version=9.2.01
  Slice11 : xbsIndex_r4/Slice  nbits=2*n_bits_out  boolean_output=off  mode=Upper Bit Location + Width  bit1=-6*n_bits_out  base1=MSB of Input  bit0=0  base0=LSB of Input  dbl_ovrd=off  block_type=slice
      settings: infoedit="Extracts a given range of bits from each input sample and presents it at the output.  The output type is ordinarily unsigned with binary point at zero, but can be Boolean when the slice is one bit wide.<P><P>Hardware notes: In hardware this block costs nothing."  block_version=9.2.01
  Slice2 : xbsIndex_r4/Slice  nbits=2*n_bits_out  boolean_output=off  mode=Upper Bit Location + Width  bit1=0  base1=MSB of Input  bit0=0  base0=LSB of Input  dbl_ovrd=off  block_type=slice
      settings: infoedit="Extracts a given range of bits from each input sample and presents it at the output.  The output type is ordinarily unsigned with binary point at zero, but can be Boolean when the slice is one bit wide.<P><P>Hardware notes: In hardware this block costs nothing."  block_version=9.2.01
  Slice{3..4,7,9} (4 alike) : xbsIndex_r4/Slice  nbits=2*n_bits  boolean_output=off  mode=Upper Bit Location + Width  bit1=-2*n_bits  base1=MSB of Input  bit0=0  base0=LSB of Input  dbl_ovrd=off  block_type=slice
      Slice3 settings: infoedit="Extracts a given range of bits from each input sample and presents it at the output.  The output type is ordinarily unsigned with binary point at zero, but can be Boolean when the slice is one bit wide.<P><P>Hardware notes: In hardware this block costs nothing."  block_version=9.2.01
      Slice4 settings: infoedit="Extracts a given range of bits from each input sample and presents it at the output.  The output type is ordinarily unsigned with binary point at zero, but can be Boolean when the slice is one bit wide.<P><P>Hardware notes: In hardware this block costs nothing."  block_version=9.2.01
      Slice7 settings: infoedit="Extracts a given range of bits from each input sample and presents it at the output.  The output type is ordinarily unsigned with binary point at zero, but can be Boolean when the slice is one bit wide.<P><P>Hardware notes: In hardware this block costs nothing."  block_version=9.2.01
      Slice9 settings: block_version=9.2.01
  Slice5 : xbsIndex_r4/Slice  nbits=2*n_bits_out  boolean_output=off  mode=Upper Bit Location + Width  bit1=-2*n_bits_out  base1=MSB of Input  bit0=0  base0=LSB of Input  dbl_ovrd=off  block_type=slice
      settings: infoedit="Extracts a given range of bits from each input sample and presents it at the output.  The output type is ordinarily unsigned with binary point at zero, but can be Boolean when the slice is one bit wide.<P><P>Hardware notes: In hardware this block costs nothing."  block_version=9.2.01
  Slice8 : xbsIndex_r4/Slice  nbits=2*n_bits_out  boolean_output=off  mode=Upper Bit Location + Width  bit1=-4*n_bits_out  base1=MSB of Input  bit0=0  base0=LSB of Input  dbl_ovrd=off  block_type=slice
      settings: infoedit="Extracts a given range of bits from each input sample and presents it at the output.  The output type is ordinarily unsigned with binary point at zero, but can be Boolean when the slice is one bit wide.<P><P>Hardware notes: In hardware this block costs nothing."  block_version=9.2.01
  Terminator : Terminator
  Terminator1 : Terminator
  Terminator2 : Terminator
  cmac1 : Subsystem  Tag=cmac  AncestorBlock=casper_library_correlator/cmac  mask(cmac){acc_len=256, n_bits_a=8, bin_pt_a=7, n_bits_b=8, bin_pt_b=7, quantization=Truncate, overflow=Wrap, mult_latency=4, add_latency=3, in_latency=0, conv_latency=0, multiplier_implementation=embedded multiplier core}
      mask prompts: acc_len "Number of Accumulations"; n_bits_a "Number of bits 'a'"; bin_pt_a "Binary point 'a'"; n_bits_b "Number of bits 'b'"; bin_pt_b "Binary point 'b'"; quantization "Quantisation"; mult_latency "Multiplier Latency"; add_latency "Adder Latency"; in_latency "Input Latency"; conv_latency "Convert Latency"; multiplier_implementation "Multiplier Implementation"
      mask help: A complex multiply-accumulate block. Full precision.
      mask init: same as r2_b16a4x512f/sys0/xeng/auto_tap/dual_pol_cmac/cmac1
      mask TypeOptions quantization: Truncate | Round  (unbiased: +/- Inf) | Round  (unbiased: Even Values)
      mask TypeOptions overflow: Wrap | Saturate | Flag as error
      mask TypeOptions multiplier_implementation: behavioral HDL | standard core | embedded multiplier core
  cmac2 : Subsystem  Tag=cmac  AncestorBlock=casper_library_correlator/cmac  mask(cmac){acc_len=256, n_bits_a=8, bin_pt_a=7, n_bits_b=8, bin_pt_b=7, quantization=Truncate, overflow=Wrap, mult_latency=4, add_latency=3, in_latency=0, conv_latency=0, multiplier_implementation=embedded multiplier core}
      mask prompts: acc_len "Number of Accumulations"; n_bits_a "Number of bits 'a'"; bin_pt_a "Binary point 'a'"; n_bits_b "Number of bits 'b'"; bin_pt_b "Binary point 'b'"; quantization "Quantisation"; mult_latency "Multiplier Latency"; add_latency "Adder Latency"; in_latency "Input Latency"; conv_latency "Convert Latency"; multiplier_implementation "Multiplier Implementation"
      mask help: A complex multiply-accumulate block. Full precision.
      mask init: same as r2_b16a4x512f/sys0/xeng/auto_tap/dual_pol_cmac/cmac1
      mask TypeOptions quantization: Truncate | Round  (unbiased: +/- Inf) | Round  (unbiased: Even Values)
      mask TypeOptions overflow: Wrap | Saturate | Flag as error
      mask TypeOptions multiplier_implementation: behavioral HDL | standard core | embedded multiplier core
  cmac3 : Subsystem  Tag=cmac  AncestorBlock=casper_library_correlator/cmac  mask(cmac){acc_len=256, n_bits_a=8, bin_pt_a=7, n_bits_b=8, bin_pt_b=7, quantization=Truncate, overflow=Wrap, mult_latency=4, add_latency=3, in_latency=0, conv_latency=0, multiplier_implementation=embedded multiplier core}
      mask prompts: acc_len "Number of Accumulations"; n_bits_a "Number of bits 'a'"; bin_pt_a "Binary point 'a'"; n_bits_b "Number of bits 'b'"; bin_pt_b "Binary point 'b'"; quantization "Quantisation"; mult_latency "Multiplier Latency"; add_latency "Adder Latency"; in_latency "Input Latency"; conv_latency "Convert Latency"; multiplier_implementation "Multiplier Implementation"
      mask help: A complex multiply-accumulate block. Full precision.
      mask init: same as r2_b16a4x512f/sys0/xeng/auto_tap/dual_pol_cmac/cmac1
      mask TypeOptions quantization: Truncate | Round  (unbiased: +/- Inf) | Round  (unbiased: Even Values)
      mask TypeOptions overflow: Wrap | Saturate | Flag as error
      mask TypeOptions multiplier_implementation: behavioral HDL | standard core | embedded multiplier core
  cmac4 : Subsystem  Tag=cmac  AncestorBlock=casper_library_correlator/cmac  mask(cmac){acc_len=256, n_bits_a=8, bin_pt_a=7, n_bits_b=8, bin_pt_b=7, quantization=Truncate, overflow=Wrap, mult_latency=4, add_latency=3, in_latency=0, conv_latency=0, multiplier_implementation=embedded multiplier core}
      mask prompts: acc_len "Number of Accumulations"; n_bits_a "Number of bits 'a'"; bin_pt_a "Binary point 'a'"; n_bits_b "Number of bits 'b'"; bin_pt_b "Binary point 'b'"; quantization "Quantisation"; mult_latency "Multiplier Latency"; add_latency "Adder Latency"; in_latency "Input Latency"; conv_latency "Convert Latency"; multiplier_implementation "Multiplier Implementation"
      mask help: A complex multiply-accumulate block. Full precision.
      mask init: same as r2_b16a4x512f/sys0/xeng/auto_tap/dual_pol_cmac/cmac1
      mask TypeOptions quantization: Truncate | Round  (unbiased: +/- Inf) | Round  (unbiased: Even Values)
      mask TypeOptions overflow: Wrap | Saturate | Flag as error
      mask TypeOptions multiplier_implementation: behavioral HDL | standard core | embedded multiplier core
  acc_out : Outport
  valid_out : Outport  Port=2
  wires:
  acc_in/1 -> Slice2/1, Slice5/1, Slice8/1, Slice11/1
  a2/1 -> Slice10/1, Slice7/1, Slice4/1, Slice1/1
  a1/1 -> Slice9/1, Slice6/1, Slice3/1, Slice/1
  cmac4/1(acc_out) -> Concat/4
  cmac3/1(acc_out) -> Concat/3
  cmac2/1(acc_out) -> Concat/2
  cmac1/1(acc_out) -> Concat/1
  cmac4/2(valid_out) -> valid_out/1
  cmac3/2(valid_out) -> Terminator2/1
  cmac2/2(valid_out) -> Terminator1/1
  sync/1 -> cmac4/4(sync), cmac3/4(sync), cmac2/4(sync), cmac1/4(sync)
  Slice11/1 -> cmac4/3(acc_in)
  Slice10/1 -> cmac4/2(c+di)
  Slice9/1 -> cmac4/1(a+bi)
  Constant4/1 -> cmac3/5(valid_in)
  Slice8/1 -> cmac3/3(acc_in)
  Slice7/1 -> cmac3/2(c+di)
  Slice6/1 -> cmac3/1(a+bi)
  Constant1/1 -> cmac2/5(valid_in)
  cmac1/2(valid_out) -> Terminator/1
  valid_in/1 -> cmac4/5(valid_in)
  Concat/1 -> acc_out/1
  Slice5/1 -> cmac2/3(acc_in)
  Slice4/1 -> cmac2/2(c+di)
  Slice3/1 -> cmac2/1(a+bi)
  Slice2/1 -> cmac1/3(acc_in)
  Slice1/1 -> cmac1/2(c+di)
  Slice/1 -> cmac1/1(a+bi)
  Constant2/1 -> cmac1/5(valid_in)

== system r2_b16a4x512f/sys0/xeng/baseline_tap3/delay ==
  din : Inport
  constant : xbsIndex_r4/Constant  const=1  gui_display_data_type=Fixed-point  arith_type=Boolean  n_bits=16  bin_pt=14  preci_type=Single  exp_width=8  frac_width=24  explicit_period=on  period=1  equ=P=C  opselect=C  inp2=PCIN>>17  opr=+  inp1=P  carry=CIN  dbl_ovrd=off  block_type=constant
  counter : xbsIndex_r4/Counter  cnt_type=Count Limited  cnt_to=DelayLen - bram_latency - 1  operation=Up  start_count=0  cnt_by_val=1  arith_type=Unsigned  n_bits=8  bin_pt=0  load_pin=off  rst=off  en=off  explicit_period=on  period=1  dbl_ovrd=off  use_behavioral_HDL=off  implementation=Fabric  use_rpm=off  block_type=counter
  ram : xbsIndex_r4/Single Port RAM  depth=256  initVector=0  distributed_mem=Block RAM  write_mode=Read Before Write  rst=off  init_reg=0  en=off  latency=bram_latency  dbl_ovrd=off  optimize=Area  block_type=spram
  dout : Outport
  wires:
  counter/1 -> ram/1
  din/1 -> ram/2
  constant/1 -> ram/3
  ram/1 -> dout/1
